simulink model "KSimulator_kuka_iiwa7"  (R2023b)
settings: Solver=ode1  StartTime=0.0  StopTime=20  FixedStep=0.001  RelTol=1e-3  EnableMultiTasking=on
undefined symbols (not defined in the file or in its folder): plotRobot
CloseFcn:
  | EraseHandles
settings Model: Creator=E. Dean  LastModifiedBy=ellio
settings SolverCC: AlgebraicLoopSolver=TrustRegion
settings DataIOCC: LimitDataPoints=on  SaveFormat=Array  SignalLoggingSaveFormat=ModelDataLogs  ReturnWorkspaceOutputs=off
settings OptimizationCC: ExpressionDepthLimit=2147483647  LifeSpan=inf
settings DebuggingCC: UnderspecifiedInitializationDetection=Classic  MergeDetectMultiDrivingBlocksExec=none  SolverPrmCheckMsg=warning  FcnCallInpInsideContextMsg=warning  UnconnectedInputMsg=warning  UnconnectedOutputMsg=warning  UnconnectedLineMsg=warning  AllowSymbolicDim=off  StateNameClashWarn=warning  SFUnexpectedBacktrackingDiag=warning  SFNoUnconditionalDefaultTransitionDiag=warning  SFExecutionAtInitializationDiag=none  ArithmeticOperatorsInVariantConditions=warning
settings HardwareCC: ProdBitPerPointer=32  ProdBitPerSizeT=32  ProdBitPerPtrDiffT=32  ProdLargestAtomicFloat=None  ProdIntDivRoundTo=Undefined  ProdEndianess=Unspecified  ProdWordSize=32  ProdHWDeviceType=32-bit Generic
settings ModelReferenceCC: EnableRefExpFcnMdlSchedulingChecks=on  PropagateSignalLabelsOutOfModel=off
settings SFSimCC: SimUseLocalCustomCode=off  CustomCodeUndefinedFunction=UseInterfaceOnly
settings RTWCC: RTWUseLocalCustomCode=off  DLArmComputeVersion=19.05
settings CodeAppCC: StateflowObjectComments=on
settings GRTTargetCC: TargetLangStandard=C89/C90 (ANSI)  CombineOutputUpdateFcns=off  GRTInterface=on
settings ConfigComp: CovMetricSettings=dw  CovSaveCumulativeToWorkspaceVar=on  CovSaveSingleToWorkspaceVar=on  CovExternalEMLEnable=off  CovSFcnEnable=off

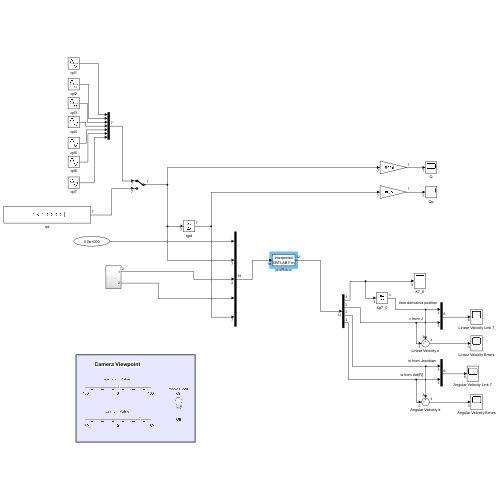
[thumbnail: Simulink's stored preview of the top-level diagram]
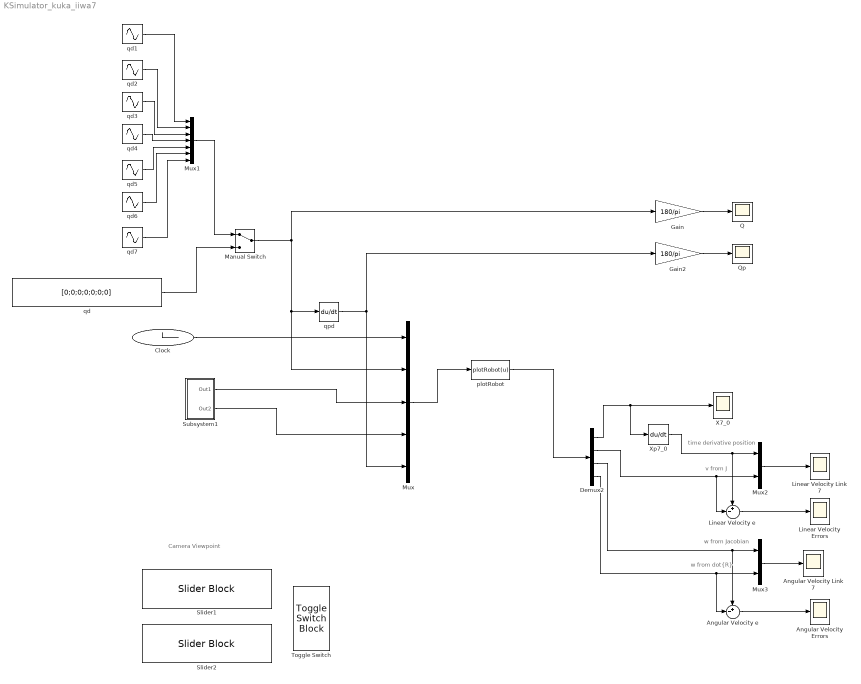
== system KSimulator_kuka_iiwa7 ==
  note: time derivative position
  note: v from J
  note: w from dot{R}
  note: w from Jacobian
  note: Camera Viewpoint
  Angular Velocity Errors : Scope
  Angular Velocity Link 7 : Scope
  Angular Velocity e : Sum  Inputs=+-|
  Clock : Clock
  Demux2 : Demux
  Gain : Gain  Gain=180/pi
  Gain2 : Gain  Gain=180/pi
  Linear Velocity Errors : Scope
  Linear Velocity Link 7 : Scope
  Linear Velocity e : Sum  Inputs=+-|
  Manual Switch : ManualSwitch
  Mux : Mux  Inputs=5
  Mux1 : Mux  Inputs=7
  Mux2 : Mux  Inputs=2
  Mux3 : Mux  Inputs=2
  Q : Scope
  Qp : Scope
  Slider1 : SliderBlock  ScaleMin=-180  ScaleMax=180  TickInterval=180
  Slider2 : SliderBlock  ScaleMin=-180  ScaleMax=180  TickInterval=180
  Subsystem1 : Subsystem
  Toggle Switch : ToggleSwitchBlock
      settings: Values={{'Off', 'On'}, [0 1]}
  X7_0 : Scope
  Xp7_0 : Derivative
  plotRobot : MATLABFcn  MATLABFcn=plotRobot(u)  OutputDimensions=12
  qd : Constant  Value=[0;0;0;0;0;0;0]
  qd1 : Sin  SampleTime=0
  qd2 : Sin  Amplitude=0.5  Bias=0.3  Frequency=0.75  SampleTime=0
  qd{3..7} (5 alike) : Sin  Amplitude=pi  Frequency=0.5  SampleTime=0
  qpd : Derivative
  wires:
  Mux/1 -> plotRobot/1
  qd1/1 -> Mux1/1
  qd2/1 -> Mux1/2
  qd3/1 -> Mux1/3
  Mux1/1 -> Manual Switch/1
  qpd/1 -> Gain2/1, Mux/5
  plotRobot/1 -> Demux2/1
  Demux2/1 -> Xp7_0/1, X7_0/1
  Mux2/1 -> Linear Velocity Link 7/1
  Xp7_0/1 -> Mux2/1, Linear Velocity e/1
  Demux2/2 -> Linear Velocity e/2, Mux2/2
  qd/1 -> Manual Switch/2
  Mux3/1 -> Angular Velocity Link 7/1
  Demux2/3 -> Angular Velocity e/1, Mux3/1
  Demux2/4 -> Angular Velocity e/2, Mux3/2
  Clock/1 -> Mux/1
  Manual Switch/1 -> Gain/1, Mux/2, qpd/1
  Subsystem1/1(Out1) -> Mux/3
  Subsystem1/2(Out2) -> Mux/4
  qd4/1 -> Mux1/4
  Linear Velocity e/1 -> Linear Velocity Errors/1
  Angular Velocity e/1 -> Angular Velocity Errors/1
  Gain/1 -> Q/1
  Gain2/1 -> Qp/1
  qd5/1 -> Mux1/5
  qd6/1 -> Mux1/6
  qd7/1 -> Mux1/7

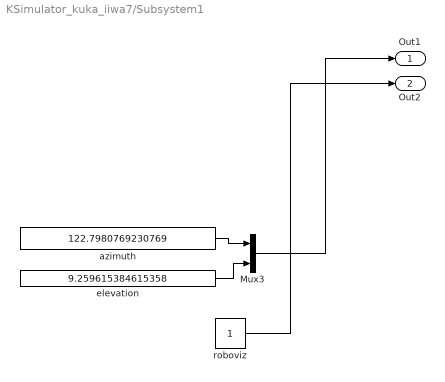
== system KSimulator_kuka_iiwa7/Subsystem1 ==
  Mux3 : Mux  Inputs=2
  azimuth : Constant  Value=122.7980769230769
  elevation : Constant  Value=9.259615384615358
  roboviz : Constant
  Out1 : Outport
  Out2 : Outport  Port=2
  wires:
  azimuth/1 -> Mux3/1
  roboviz/1 -> Out2/1
  elevation/1 -> Mux3/2
  Mux3/1 -> Out1/1
